simulink model "simulacija_regulacije_nova"  (R2015b)
settings: Solver=FixedStepAuto  StartTime=0.0  StopTime=1000  RelTol=1e-3
undefined symbols (not defined in the file): K1, K2, tau1, tau2
settings Model: Creator=Elma  LastModifiedBy=Elma

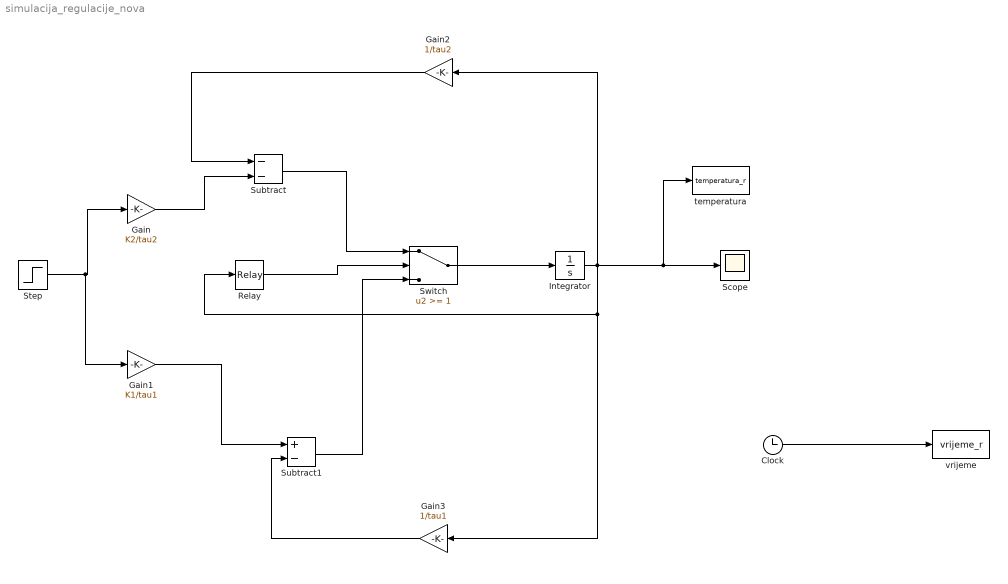
== system simulacija_regulacije_nova ==
  Clock : Clock
  Gain : Gain  Gain=K2/tau2
  Gain1 : Gain  Gain=K1/tau1
  Gain2 : Gain  Gain=1/tau2
  Gain3 : Gain  Gain=1/tau1
  Integrator : Integrator
  Relay : Relay  OnSwitchValue=97  OffSwitchValue=94
  Scope : Scope
  Step : Step  SampleTime=0
  Subtract : Sum  Inputs=--
  Subtract1 : Sum  Inputs=+-
  Switch : Switch  Threshold=1
  temperatura : ToWorkspace  VariableName=temperatura_r  SaveFormat=Timeseries  SampleTime=-1
  vrijeme : ToWorkspace  VariableName=vrijeme_r  SaveFormat=Timeseries  SampleTime=-1
  wires:
  Step/1 -> Gain1/1, Gain/1
  Gain/1 -> Subtract/2
  Gain2/1 -> Subtract/1
  Subtract/1 -> Switch/1
  Switch/1 -> Integrator/1
  Integrator/1 -> Gain3/1, Relay/1, temperatura/1, Scope/1, Gain2/1
  Relay/1 -> Switch/2
  Gain1/1 -> Subtract1/1
  Gain3/1 -> Subtract1/2
  Subtract1/1 -> Switch/3
  Clock/1 -> vrijeme/1
